simulink model "Transitions_Conditions_States"  (R2026a)
settings: Solver=VariableStepAuto
StartFcn:
  | learning.simulink.modelCallbacks.startFunction(gcs);
StopFcn:
  | learning.simulink.modelCallbacks.stopFunction(gcs);
model workspace (MAT data in the model file):
  courseObject.course = 'stateflow'
  courseObject.chapter = 3
  courseObject.lesson = 2
  courseObject.section = 1
  courseObject.task = 1
libraries: SignalEditorBlockLib x1, signalChecks x1
CloseFcn:
  | learning.simulink.cleanupOnlineTraining;learning.simulink.Application.getInstance().dduxLogMatlabEvent("ModelClosed");
Description:
  | TrainingCourseModel
settings Model: Creator=PC  LastModifiedBy=PC

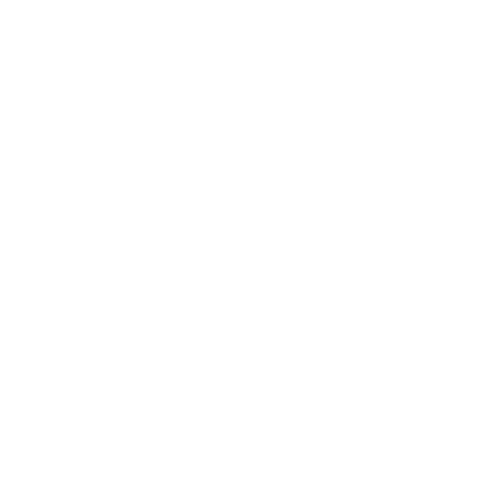
[thumbnail: Simulink's stored preview of the top-level diagram]
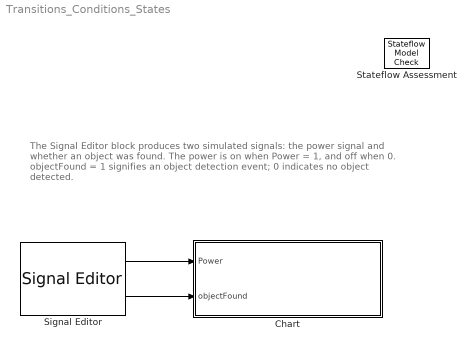
== system Transitions_Conditions_States ==
  note: The Signal Editor block produces two simulated signals: the power signal and whether an object was found.
      | The power is on when Power = 1, and off when 0.
      | objectFound = 1 signifies an object detection event; 0 indicates no object detected.
  Chart : Stateflow chart  TreatAsAtomicUnit=on
  Signal Editor : SignalEditorBlockLib/Signal Editor  FileName=objectTrackerTestSignal.mat  ActiveScenario=Scenario  ActiveSignal=Power  IsBus=off  OutputBusObjectStr=Bus: BusObject  SampleTime=0.5  Interpolate=off  ZeroCross=off  OutputAfterFinalValue=Setting to zero  Unit=inherit  PreserveSignalName=on  ApplySigPropsToAllScenarios=on  ApplySigPropsToAllSignals=off  SignalPropertySource=Dialog parameters
  Stateflow Assessment : signalChecks/Stateflow Model Check  mlfunc='LearningApplication.gradeStateflowTask'  flags='transitionExOrder'  startInChart=true  lesson=0  task=6  pass=-1
      settings: AttributesFormatString=|
      | No input required
      | for this task
  wires:
  Signal Editor/2 -> Chart/2(objectFound)
  Signal Editor/1 -> Chart/1(Power)

== stateflow chart Transitions_Conditions_States/Chart ==
  state Off
  state Seeking
  state Tracking
  (default) -> Off
  Off -> Seeking : [Power == 1]
  Seeking -> Off [order 1] : [Power == 0]
  (junction 30) -> Off
  Tracking -> Seeking [order 2] : [objectFound == 0]
  Seeking -> Tracking [order 2] : [objectFound ==1]
  Tracking -> (junction 30) [order 1] : [Power == 0]
  data: Power input; objectFound input
